simulink model "gnc"  (R2026a)
settings: Solver=VariableStepAuto
libraries: dspmathops x1
settings Model: Creator=aayush  LastModifiedBy=aayush

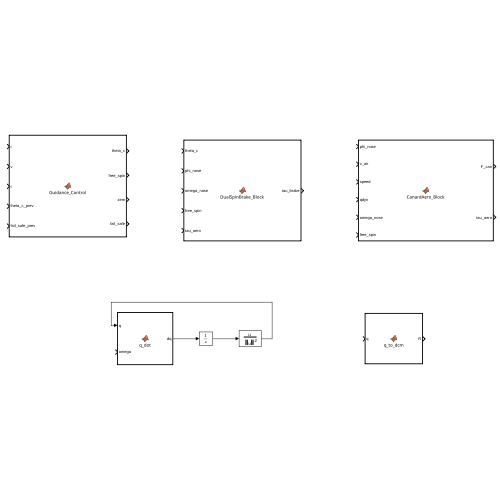
[thumbnail: Simulink's stored preview of the top-level diagram]
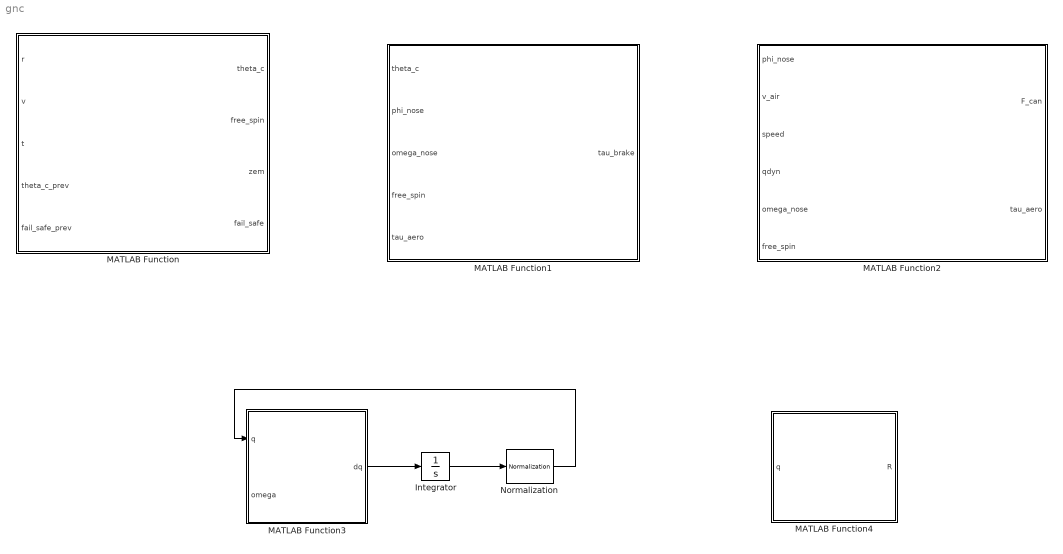
== system gnc ==
  Integrator : Integrator
  MATLAB Function : MATLAB Function  TreatAsAtomicUnit=on
  MATLAB Function1 : MATLAB Function  TreatAsAtomicUnit=on
  MATLAB Function2 : MATLAB Function  TreatAsAtomicUnit=on
  MATLAB Function3 : MATLAB Function  TreatAsAtomicUnit=on
  MATLAB Function4 : MATLAB Function  TreatAsAtomicUnit=on
  Normalization : dspmathops/Normalization  NormType=Squared 2-norm  Bias=1e-10  NormOver=Each column  Dimension=1  roundingMode=Floor  overflowMode=off  accumDataTypeStr=Inherit: Same as product output  accumLastDataTypeStr=Inherit: Same as product output  outputDataTypeStr=Inherit: Same as product output  outputMin=[]  outputMax=[]  outputLastDataTypeStr=Inherit: Same as product output
  wires:
  MATLAB Function3/1(dq) -> Integrator/1
  Integrator/1 -> Normalization/1
  Normalization/1 -> MATLAB Function3/1(q)

== matlab function gnc/MATLAB Function1 ==
  data: theta_c input; tau_brake output; phi_nose input; omega_nose input; free_spin input; tau_aero input
function tau_brake = DualSpinBrake_Block(theta_c, phi_nose, omega_nose, free_spin, tau_aero)
coder.extrinsic('init_pgk_params');
params = init_pgk_params();

% Alternator load (simplified)
tau_alt = 0; 

if free_spin
    % Free-spin: brake off, only aero/alternator load
    tau_cmd = tau_aero + tau_alt;
else
    % Hold mode: drive omega_nose to 0 and phi_nose to theta_c
    err_phi = wrapToPi(theta_c - phi_nose);
    tau_cmd = 0.15 * tau_aero + tau_alt ...
        - params.K_brake * omega_nose ...
        + params.K_phi_hold * err_phi;
end
tau_brake = max(-params.brake_torque_max, min(params.brake_torque_max, tau_cmd));
end

== matlab function gnc/MATLAB Function ==
  data: r input; theta_c output; v input; t input; theta_c_prev input; fail_safe_prev input; free_spin output; zem output; fail_safe output
function [theta_c, free_spin, zem, fail_safe] = Guidance_Control(r, v, t, theta_c_prev, fail_safe_prev)
    % Load params from workspace
    coder.extrinsic('init_pgk_params');
    params = init_pgk_params();
    target = params.target;
    
    % 1. Impact Predictor (Simplified constant Cd)
    dt_pred = params.predictor_dt;
    rr = r; vv = v;
    tgo = 0;
    while rr(3) > 0 && tgo < 45.0
        speed = norm(vv);
        if speed > 1.0
            a_drag = -0.27 * 0.5 * params.rho0 * speed^2 * params.ref_area / params.mass * (vv/speed);
        else
            a_drag = [0;0;0];
        end
        a = a_drag + [0; 0; -params.g0]; % F_can_est omitted for simplicity in predictor
        vv = vv + a * dt_pred;
        rr = rr + vv * dt_pred;
        tgo = tgo + dt_pred;
    end
    impact = rr; impact(3) = 0;
    
    % 2. ZEM Calculation
    zem_vec = target(1:2) - impact(1:2);
    zem = norm(zem_vec);
    
    % 3. Fail-Safe Logic
    fail_safe = fail_safe_prev;
    if t >= params.fail_safe_check_time && ~fail_safe_prev
        if zem > params.fail_safe_miss * 8.0
            fail_safe = true;
        end
    end
    
    % 4. Mode & Theta_C Command
    if t < params.arm_time || fail_safe || zem < params.zem_deadband
        free_spin = true;
        theta_c = theta_c_prev;
    else
        free_spin = false;
        desired = atan2(zem_vec(2), zem_vec(1)) + params.guidance_phase_deg;
        err = wrapToPi(desired - theta_c_prev);
        max_rate = deg2rad(params.max_slew_rate_deg);
        rate = max(-max_rate, min(max_rate, params.K_orient * err));
        alpha = params.control_dt / (params.orientation_slew_tau + params.control_dt);
        theta_c = mod(theta_c_prev + alpha * rate * params.orientation_slew_tau, 2*pi);
    end
end

== matlab function gnc/MATLAB Function2 ==
  data: phi_nose input; v_air input; speed input; qdyn input; F_can output; omega_nose input; free_spin input; tau_aero output
function [F_can, tau_aero] = CanardAero_Block(phi_nose, v_air, speed, qdyn, omega_nose, free_spin)
    coder.extrinsic('init_pgk_params');
    params = init_pgk_params();
    
    if free_spin || speed < params.canard_min_speed || abs(omega_nose) >= 40.0
        F_can = [0; 0; 0];
        tau_aero = 0;
        return;
    end
    
    % Direction
    c_phi = cos(phi_nose); s_phi = sin(phi_nose);
    desired = [c_phi; s_phi; 0];
    vhat = v_air / (speed + 1e-9);
    force_dir = desired - dot(desired, vhat) * vhat;
    n = norm(force_dir);
    if n < 1e-6
        F_can = [0; 0; 0]; tau_aero = 0; return;
    end
    force_dir = force_dir / n;
    
    % Magnitude
    CN0 = params.canard_Cl_max * params.canard_authority * params.canard_area / params.ref_area;
    Fmag = CN0 * qdyn * params.ref_area;
    Fmag = min(Fmag, params.canard_a_max * params.mass);
    
    F_can = Fmag * force_dir;
    
    % Aero de-spin torque on nose
    tau_aero = -params.aero_despin_coeff * qdyn * sign(omega_nose) * min(abs(omega_nose)/80.0, 1.0);
end

== matlab function gnc/MATLAB Function3 ==
  data: q input; dq output; omega input
function dq = q_dot(q, omega)
    p = omega(1); qr = omega(2); r = omega(3);
    Om = [0, -p, -qr, -r;
          p,  0,  r, -qr;
          qr, -r, 0,  p;
          r,  qr, -p, 0];
    dq = 0.5 * (Om * q);
end

== matlab function gnc/MATLAB Function4 ==
  data: q input; R output
function R = q_to_dcm(q)
    w = q(1); x = q(2); y = q(3); z = q(4);
    R = [1-2*(y^2+z^2), 2*(x*y-w*z), 2*(x*z+w*y);
         2*(x*y+w*z), 1-2*(x^2+z^2), 2*(y*z-w*x);
         2*(x*z-w*y), 2*(y*z+w*x), 1-2*(x^2+y^2)];
end
